simulink model "foc_gpio_can_probe"  (R2023a)
settings: Solver=FixedStepDiscrete  StartTime=0.0  StopTime=inf  FixedStep=0.00025  RelTol=1e-3  EnableMultiTasking=on
libraries: c2838xlib x3
settings Model: ExtModeTrigDuration=8  Creator=Student  LastModifiedBy=Student
settings OptimizationCC: DefaultUnderspecifiedDataType=single  EnhancedBackFolding=on  PassReuseOutputArgsAs=Individual arguments  MaxStackSize=1024  OptimizeBlockOrder=speed  DifferentSizesBufferReuse=on  OptimizationCustomize=off  DenormalBehavior=FlushToZero  EfficientTunableParamExpr=on
settings DebuggingCC: ParameterTunabilityLossMsg=error
settings HardwareCC: ProdBitPerChar=16  ProdBitPerInt=16  ProdBitPerPointer=32  ProdBitPerSizeT=32  ProdBitPerPtrDiffT=32  ProdLargestAtomicInteger=Integer  ProdLargestAtomicFloat=None  ProdWordSize=16  ProdLongLongMode=on  ProdHWDeviceType=Texas Instruments->C2000  HardwareBoardFeatureSet=SoCBlockset
settings ModelReferenceCC: ModelReferenceNumInstancesAllowed=Single
settings SFSimCC: MATLABDynamicMemAlloc=off
settings RTWCC: Description=Embedded Coder  SystemTargetFile=ert.tlc  HardwareBoard=TI F2838x  TemplateMakefile=ert_default_tmf  Toolchain=Texas Instruments Code Composer Studio - EABI (C2000)
settings CodeAppCC: ForceParamTrailComments=on  IgnoreCustomStorageClasses=off  OperatorAnnotations=on  SimulinkDataObjDesc=on  SFDataObjDesc=on  InsertBlockDesc=on
settings ERTTargetCC: CodeReplacementLibrary=TI C28x  ExtModeTransport=4  ExtModeStaticAlloc=on  ExtModeAutomaticAllocSize=off  ExtModeStaticAllocSize=10000  ExtModeMexFile=ext_xcp  ExtModeIntrfLevel=Level2 - Open

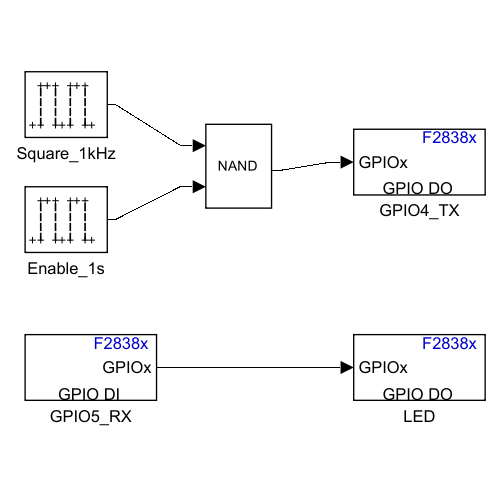
[thumbnail: Simulink's stored preview of the top-level diagram]
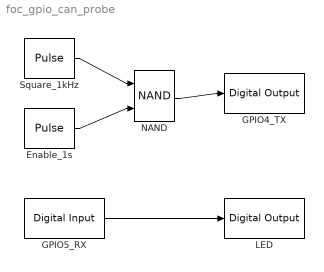
== system foc_gpio_can_probe ==
  Enable_1s : DiscretePulseGenerator  Period=8000  PulseWidth=4000  SampleTime=0.00025
  GPIO4_TX : c2838xlib/Digital Output  GPIO_Number=GPIO0~GPIO7  GPIO_Bit0=off  GPIO_BIT0_Toggle=off  GPIO_Bit1=off  GPIO_BIT1_Toggle=off  GPIO_Bit2=off  GPIO_BIT2_Toggle=off  GPIO_Bit3=off  GPIO_BIT3_Toggle=off  GPIO_Bit4=on  GPIO_BIT4_Toggle=off  GPIO_Bit5=off  GPIO_BIT5_Toggle=off  GPIO_Bit6=off  GPIO_BIT6_Toggle=off  GPIO_Bit7=off  GPIO_BIT7_Toggle=off
  GPIO5_RX : c2838xlib/Digital Input  GPIO_Number=GPIO0~GPIO7  GPIO_Bit0=off  GPIO_Bit1=off  GPIO_Bit2=off  GPIO_Bit3=off  GPIO_Bit4=off  GPIO_Bit5=on  GPIO_Bit6=off  GPIO_Bit7=off  sampleTime=0.01  dataType=auto  GPIO_Bit0_Qualification=Sync to SYSCLKOUT  GPIO_Bit1_Qualification=Sync to SYSCLKOUT  GPIO_Bit2_Qualification=Sync to SYSCLKOUT  GPIO_Bit3_Qualification=Sync to SYSCLKOUT  GPIO_Bit4_Qualification=Sync to SYSCLKOUT  GPIO_Bit5_Qualification=Sync to SYSCLKOUT  GPIO_Bit6_Qualification=Sync to SYSCLKOUT  GPIO_Bit7_Qualification=Sync to SYSCLKOUT  Qualification_Period=-1
  LED : c2838xlib/Digital Output  GPIO_Number=GPIO56~GPIO63  GPIO_Bit0=on  GPIO_BIT0_Toggle=off  GPIO_Bit1=off  GPIO_BIT1_Toggle=off  GPIO_Bit2=off  GPIO_BIT2_Toggle=off  GPIO_Bit3=off  GPIO_BIT3_Toggle=off  GPIO_Bit4=off  GPIO_BIT4_Toggle=off  GPIO_Bit5=off  GPIO_BIT5_Toggle=off  GPIO_Bit6=off  GPIO_BIT6_Toggle=off  GPIO_Bit7=off  GPIO_BIT7_Toggle=off
  NAND : Logic  Operator=NAND  AllPortsSameDT=off  OutDataTypeStr=boolean
  Square_1kHz : DiscretePulseGenerator  Period=4  PulseWidth=2  SampleTime=0.00025
  wires:
  Square_1kHz/1 -> NAND/1
  Enable_1s/1 -> NAND/2
  NAND/1 -> GPIO4_TX/1
  GPIO5_RX/1 -> LED/1
